simulink model "esc_motorS"  (R2025b)
settings: Solver=FixedStepDiscrete  StartTime=0.0  StopTime=inf  FixedStep=0.05  RelTol=1e-3
undefined symbols (not defined in the file or in its folder): escSerial
settings Model: Creator=FOFIEVIGOLBRYAN  LastModifiedBy=FOFIEVIGOLBRYAN

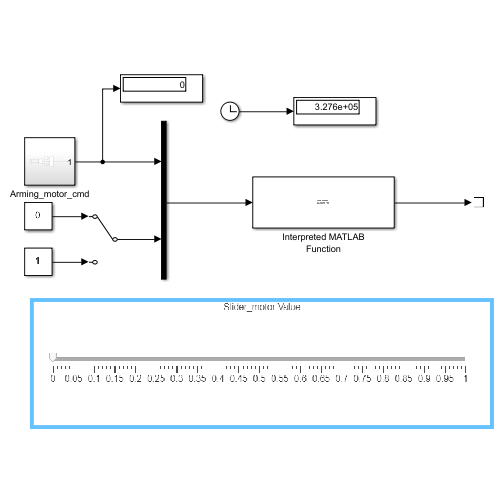
[thumbnail: Simulink's stored preview of the top-level diagram]
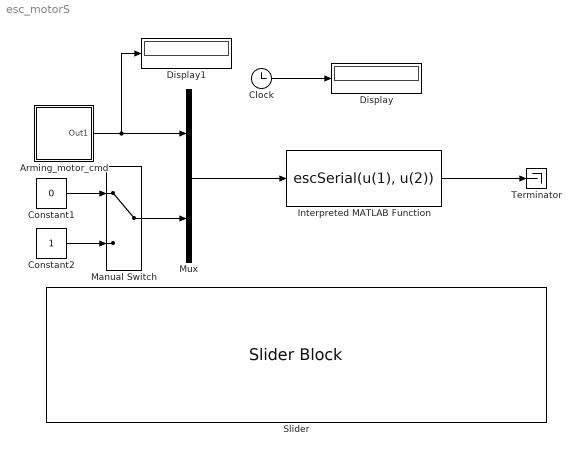
== system esc_motorS ==
  Arming_motor_cmd : Subsystem
  Clock : Clock
  Constant1 : Constant  Value=0  OutDataTypeStr=double
  Constant2 : Constant  OutDataTypeStr=double
  Display : Display
  Display1 : Display
  Interpreted MATLAB Function : MATLABFcn  MATLABFcn=escSerial(u(1), u(2))  OutputDimensions=1
  Manual Switch : ManualSwitch
  Mux : Mux  Inputs=2
  Slider : SliderBlock  ScaleMax=1
  Terminator : Terminator
  wires:
  Constant2/1 -> Manual Switch/2
  Constant1/1 -> Manual Switch/1
  Manual Switch/1 -> Mux/2
  Mux/1 -> Interpreted MATLAB Function/1
  Clock/1 -> Display/1
  Interpreted MATLAB Function/1 -> Terminator/1
  Arming_motor_cmd/1(Out1) -> Display1/1, Mux/1

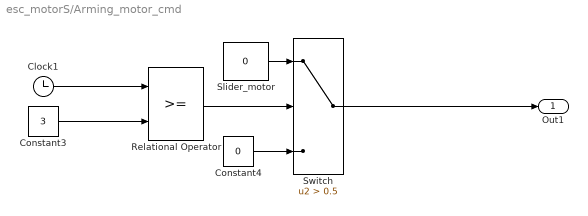
== system esc_motorS/Arming_motor_cmd ==
  Clock1 : Clock
  Constant3 : Constant  Value=3  OutDataTypeStr=double
  Constant4 : Constant  Value=0  OutDataTypeStr=double
  Relational Operator : RelationalOperator  OutDataTypeStr=boolean  RndMeth=Simplest  InputSameDT=off
  Slider_motor : Constant  Value=0  OutDataTypeStr=double
  Switch : Switch  Criteria=u2 > Threshold  Threshold=0.5  SaturateOnIntegerOverflow=off  InputSameDT=off
  Out1 : Outport
  wires:
  Constant4/1 -> Switch/3
  Constant3/1 -> Relational Operator/2
  Slider_motor/1 -> Switch/1
  Clock1/1 -> Relational Operator/1
  Switch/1 -> Out1/1
  Relational Operator/1 -> Switch/2
